simulink subsystem "pendulum_nonlinear_matlab"  (R2024b)
settings: Solver=VariableStepAuto  StartTime=0.0  StopTime=10.0  RelTol=1e-3
undefined symbols (not defined in the file): params, Ts
settings Model: Creator=dsagn  LastModifiedBy=dsagn
settings ModelReferenceCC: UpdateModelReferenceTargets=IfOutOfDate
settings SFSimCC: SimGPUStackLimitPerThread=51200
settings RTWCC: GPUStackLimitPerThread=51200  GPUComputeCapability=7.5
settings ConfigComp: CovMetricSettings=de  CovBoundaryAbsTol=1.0e-5

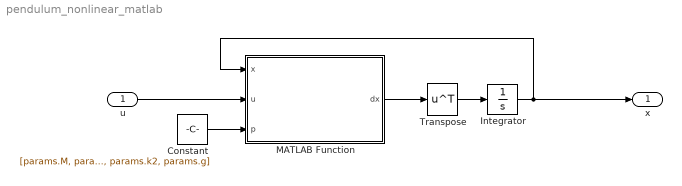
== system pendulum_nonlinear_matlab ==
  u : Inport  SampleTime=Ts
  Constant : Constant  Value=[params.M, params.m, params.l, params.k1, params.k2, params.g]  SampleTime=Ts
  Integrator : Integrator  InitialCondition=params.IC
  MATLAB Function : MATLAB Function  TreatAsAtomicUnit=on
  Transpose : Math  Operator=transpose
  x : Outport  SampleTime=Ts
  wires:
  u/1 -> MATLAB Function/2(u)
  Integrator/1 -> MATLAB Function/1(x), x/1
  MATLAB Function/1(dx) -> Transpose/1
  Transpose/1 -> Integrator/1
  Constant/1 -> MATLAB Function/3(p)

== matlab function pendulum_nonlinear_matlab/MATLAB Function ==
  data: x input; u input; dx output; p input
function dx = plant(x, u, p)
% p = [M, m, l, k1, k2, g]

    params = struct('M', p(1), 'm', p(2), 'l', p(3), 'k1', p(4), 'k2', p(5), 'g', p(6));
    dx = pendulum_cart_nl(x(:), u, params);
end
